simulink model "robot_2int"  (R2024b)
settings: Solver=VariableStepAuto  StartTime=0.0  StopTime=10.0  RelTol=1e-3
values from neighbouring files (symbols this model uses):
  A_raid = diag([500, 500])    [solve_tp1.m]
  B_raid = diag([3000, 3000])    [solve_tp1.m]
  f_d = [10; 0]    [solve_tp1.m]
  K_raid = diag([2500, 2500])    [solve_tp1.m]
  Ke_souple = diag([10^3, 0])    [solve_tp1.m]
  kp = 9*10^-2    (= 0.09)    [solve_tp1.m]
settings Model: Creator=yago.milagres-passos  LastModifiedBy=yagom

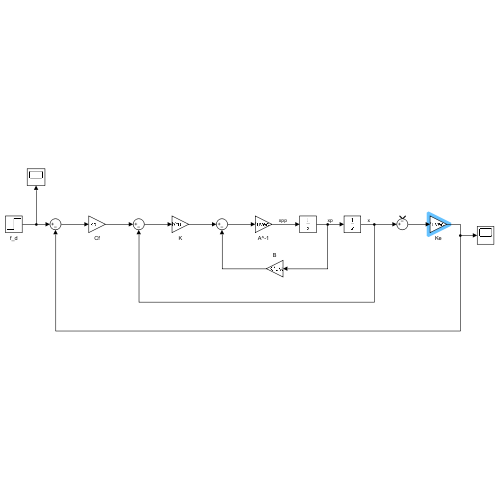
[thumbnail: Simulink's stored preview of the top-level diagram]
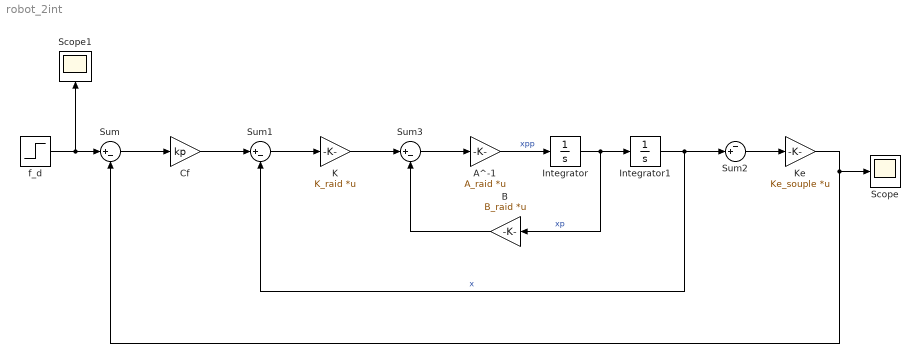
== system robot_2int ==
  A^-1 : Gain  Gain=A_raid  Multiplication=Matrix(K*u) (u vector)
  B : Gain  Gain=B_raid  Multiplication=Matrix(K*u) (u vector)
  Cf : Gain  Gain=kp
  Integrator : Integrator
  Integrator1 : Integrator
  K : Gain  Gain=K_raid  Multiplication=Matrix(K*u)
  Ke : Gain  Gain=Ke_souple  Multiplication=Matrix(K*u) (u vector)
  Scope : Scope
  Scope1 : Scope
  Sum : Sum  Inputs=|+-
  Sum1 : Sum  Inputs=|+-
  Sum2 : Sum  Inputs=-+|
  Sum3 : Sum  Inputs=|+-
  f_d : Step  After=f_d  SampleTime=0
  wires:
  f_d/1 -> Scope1/1, Sum/1
  Sum/1 -> Cf/1
  Cf/1 -> Sum1/1
  Sum1/1 -> K/1
  A^-1/1 -> Integrator/1  "xpp"
  Integrator/1 -> B/1, Integrator1/1  "xp"
  Integrator1/1 -> Sum1/2, Sum2/2  "x"
  Sum2/1 -> Ke/1
  K/1 -> Sum3/1
  Sum3/1 -> A^-1/1
  B/1 -> Sum3/2
  Ke/1 -> Sum/2, Scope/1
